simulink model "sparrow_albatros_spec_withgpio_bram"  (R2021a)
settings: Solver=VariableStepDiscrete  StartTime=0.0  StopTime=200000  RelTol=1e-3
undefined symbols (not defined in the file): pfb_coeff_gen_calc
libraries: xbsIndex_r4 x5629, casper_library_misc x33, casper_library_delays x28, xps_library x10, simulink x8, xbsReplacements_r4 x2
(part 5 of 85)

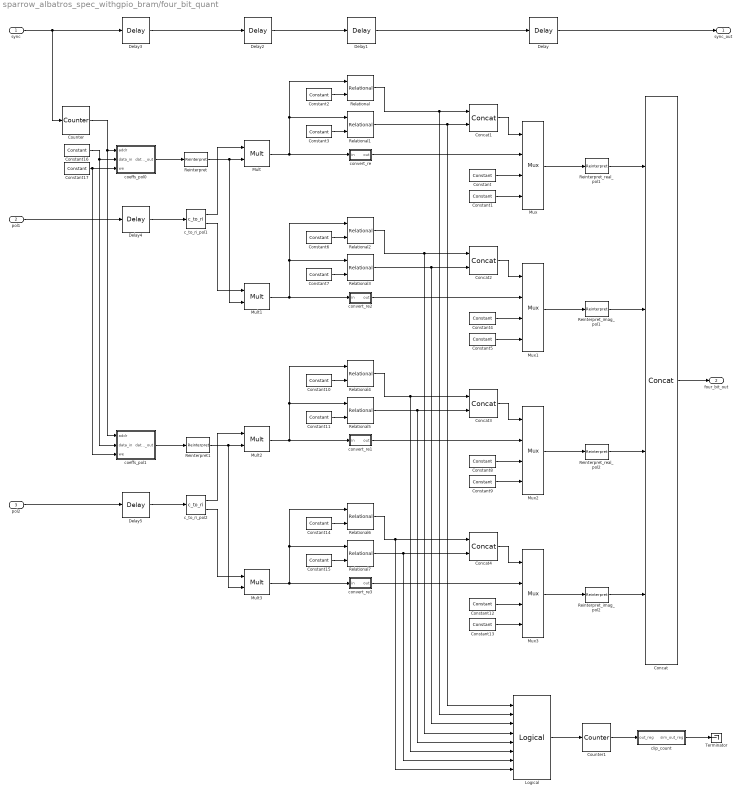
== system sparrow_albatros_spec_withgpio_bram/four_bit_quant ==
  sync : Inport
  pol1 : Inport  Port=2
  pol2 : Inport  Port=3
  Concat : xbsIndex_r4/Concat  num_inputs=4  dbl_ovrd=off  block_type=concat
  Concat{1..4} (4 alike) : xbsIndex_r4/Concat  num_inputs=2  dbl_ovrd=off  block_type=concat
  Constant{,4,8,12} (4 alike) : xbsIndex_r4/Constant  const=7/8  gui_display_data_type=Fixed-point  arith_type=Signed (2's comp)  n_bits=4  bin_pt=3  preci_type=Single  exp_width=8  frac_width=24  explicit_period=on  period=1  equ=P=C  opselect=C  inp2=PCIN>>17  opr=+  inp1=P  carry=CIN  dbl_ovrd=off  block_type=constant
  Constant{1,5,9,13} (4 alike) : xbsIndex_r4/Constant  const=-7/8  gui_display_data_type=Fixed-point  arith_type=Signed (2's comp)  n_bits=4  bin_pt=3  preci_type=Single  exp_width=8  frac_width=24  explicit_period=on  period=1  equ=P=C  opselect=C  inp2=PCIN>>17  opr=+  inp1=P  carry=CIN  dbl_ovrd=off  block_type=constant
  Constant{2,6,10,14} (4 alike) : xbsIndex_r4/Constant  const=-7/8  gui_display_data_type=Fixed-point  arith_type=Signed (2's comp)  n_bits=18  bin_pt=17  preci_type=Single  exp_width=8  frac_width=24  explicit_period=on  period=1  equ=P=C  opselect=C  inp2=PCIN>>17  opr=+  inp1=P  carry=CIN  dbl_ovrd=off  block_type=constant
  Constant{3,7,11,15} (4 alike) : xbsIndex_r4/Constant  const=7/8  gui_display_data_type=Fixed-point  arith_type=Signed (2's comp)  n_bits=18  bin_pt=17  preci_type=Single  exp_width=8  frac_width=24  explicit_period=on  period=1  equ=P=C  opselect=C  inp2=PCIN>>17  opr=+  inp1=P  carry=CIN  dbl_ovrd=off  block_type=constant
  Constant16 : xbsIndex_r4/Constant  const=0  gui_display_data_type=Fixed-point  arith_type=Signed (2's comp)  n_bits=32  bin_pt=0  preci_type=Single  exp_width=8  frac_width=24  explicit_period=on  period=1  equ=P=C  opselect=C  inp2=PCIN>>17  opr=+  inp1=P  carry=CIN  dbl_ovrd=off  block_type=constant
  Constant17 : xbsIndex_r4/Constant  const=0  gui_display_data_type=Boolean  arith_type=Boolean  n_bits=16  bin_pt=14  preci_type=Single  exp_width=8  frac_width=24  explicit_period=on  period=1  equ=P=C  opselect=C  inp2=PCIN>>17  opr=+  inp1=P  carry=CIN  dbl_ovrd=off  block_type=constant
  Counter : xbsIndex_r4/Counter  cnt_type=Free Running  cnt_to=50  operation=Up  start_count=0  cnt_by_val=1  arith_type=Unsigned  n_bits=11  bin_pt=0  load_pin=off  rst=on  en=off  explicit_period=on  period=1  use_behavioral_HDL=off  implementation=Fabric  dbl_ovrd=off  block_type=counter
  Counter1 : xbsIndex_r4/Counter  cnt_type=Free Running  cnt_to=Inf  operation=Up  start_count=0  cnt_by_val=1  arith_type=Unsigned  n_bits=32  bin_pt=0  load_pin=off  rst=off  en=on  explicit_period=on  period=1  use_behavioral_HDL=off  implementation=Fabric  dbl_ovrd=off  block_type=counter
  Delay{,3..5} (4 alike) : xbsIndex_r4/Delay  rst=off  infoeditControl=Selection of Reset will increase slice count due to use of real FFs and instead of SRLs  en=off  latency=1  reg_retiming=off  dbl_ovrd=off  block_type=delay
  Delay1 : xbsIndex_r4/Delay  rst=off  infoeditControl=Selection of Reset will increase slice count due to use of real FFs and instead of SRLs  en=off  latency=2  reg_retiming=off  dbl_ovrd=off  block_type=delay
  Delay2 : xbsIndex_r4/Delay  rst=off  infoeditControl=Selection of Reset will increase slice count due to use of real FFs and instead of SRLs  en=off  latency=3  reg_retiming=off  dbl_ovrd=off  block_type=delay
  Logical : xbsIndex_r4/Logical  logical_function=OR  inputs=8  en=off  latency=1  precision=Full  arith_type=Unsigned  n_bits=16  bin_pt=0  align_bp=on  dbl_ovrd=off  block_type=logical
  Mult{,1..3} (4 alike) : xbsIndex_r4/Mult  precision=Full  arith_type="Signed  (2's comp)"  n_bits=16  bin_pt=14  quantization=Truncate  overflow=Wrap  en=off  latency=3  use_behavioral_HDL=off  opt=Speed  use_embedded=on  optimum_pipeline=off  pipeline=on  dbl_ovrd=off  use_rpm=on  placement_style=Triangular  block_type=mult
  Mux{,1..3} (4 alike) : xbsIndex_r4/Mux  inputs=3  en=off  latency=1  precision=Full  arith_type=Unsigned  n_bits=16  bin_pt=14  quantization=Truncate  overflow=Wrap  dbl_ovrd=off  block_type=mux
  Reinterpret : xbsIndex_r4/Reinterpret  force_arith_type=on  arith_type="Signed  (2's comp)"  force_bin_pt=on  bin_pt=15  block_type=reinterpret
  Reinterpret1 : xbsIndex_r4/Reinterpret  force_arith_type=on  arith_type="Signed  (2's comp)"  force_bin_pt=on  bin_pt=15  block_type=reinterpret
  Reinterpret_imag_pol1 : xbsIndex_r4/Reinterpret  force_arith_type=on  arith_type=Unsigned  force_bin_pt=on  bin_pt=0  block_type=reinterpret
  Reinterpret_imag_pol2 : xbsIndex_r4/Reinterpret  force_arith_type=on  arith_type=Unsigned  force_bin_pt=on  bin_pt=0  block_type=reinterpret
  Reinterpret_real_pol1 : xbsIndex_r4/Reinterpret  force_arith_type=on  arith_type=Unsigned  force_bin_pt=on  bin_pt=0  block_type=reinterpret
  Reinterpret_real_pol2 : xbsIndex_r4/Reinterpret  force_arith_type=on  arith_type=Unsigned  force_bin_pt=on  bin_pt=0  block_type=reinterpret
  Relational{,2,4,6} (4 alike) : xbsIndex_r4/Relational  mode=a<b  op_type=Bool  en=off  latency=2  dbl_ovrd=off  block_type=relational
  Relational{1,3,5,7} (4 alike) : xbsIndex_r4/Relational  mode=a>b  op_type=Bool  en=off  latency=2  dbl_ovrd=off  block_type=relational
  Terminator : Terminator
  c_to_ri_pol1 : casper_library_misc/c_to_ri  n_bits=24  bin_pt=23
      settings: AttributesFormatString=24_23 r/i  SourceProductName=CASPER DSP Blockset
  c_to_ri_pol2 : casper_library_misc/c_to_ri  n_bits=24  bin_pt=23
      settings: AttributesFormatString=24_23 r/i  SourceProductName=CASPER DSP Blockset
  clip_count : Subsystem  Tag=xps:sw_reg  AncestorBlock=xps_library/Memory/software_register  mask(swreg){io_dir=To Processor, io_delay=0, init_val=0, sample_period=1, names=reg, bitwidths=32, bin_pts=0, arith_types=0, sim_port=on, show_format=on}
      mask prompts: io_dir "I/O direction"; io_delay "I/O delay"; init_val "Initial Value"; sample_period "Sample period"; names "Bitfield names [msb...lsb]"; bitwidths "Bitfield widths"; bin_pts "Bitfield binary pts"; arith_types "Bitfield types, ufix=0, fix=1, bool=2"; sim_port "Provide sim input/output?"; show_format "Print format string?"
      mask help: A 32-bit software-accessible register. Can be divided into bitfields of varying widths and types using the fields in the block mask.
      mask init:
      | swreg_init(gcb)
      settings: AttributesFormatString=1output:uf32.0 = 32 bits
      mask TypeOptions io_dir: To Processor | From Processor
      mask Callback io_dir:
      | mask_enables = get_param(gcb, 'MaskEnables');
      | mask_names = get_param(gcb, 'MaskNames');
      | if strcmp(get_param(gcb, 'io_dir'), 'To Processor'),
      |     mask_enables{ismember(mask_names, 'sample_period')} = 'off';
      | else
      |     mask_enables{ismember(mask_names, 'sample_period')} = 'on';
      | end
      | set_param(gcb, 'MaskEnables', mask_enables);
      mask DialogControl ParameterTabVar0 Prompt: Setup
  coeffs_pol0 : Subsystem  Tag=xps:bram  AncestorBlock=xps_library/Memory/shared_bram  mask{arith_type=Unsigned, addr_width=11, data_width=32, reg_prim_output=off, reg_core_output=off, optimization=Minimum_Area, data_bin_pt=0, init_vals=ones(1,2048)*(2^31), sample_rate=1}
      mask prompts: arith_type "Output Data Type"; addr_width "Address width"; data_width "Data Width"; reg_prim_output "Register Primitive Output"; reg_core_output "Register Core Output"; data_bin_pt "Data Binary Point"; init_vals "Initial values (simulation only)"; sample_rate "Sample rate"
      mask init:
      | shared_bram_mask;
      mask TypeOptions arith_type: Unsigned | Signed  (2's comp)
      mask TypeOptions data_width: 8 | 16 | 32 | 64 | 128
      mask TypeOptions optimization: Minimum_Area | Low_Power
  coeffs_pol1 : Subsystem  Tag=xps:bram  AncestorBlock=xps_library/Memory/shared_bram  mask{arith_type=Unsigned, addr_width=11, data_width=32, reg_prim_output=off, reg_core_output=off, optimization=Minimum_Area, data_bin_pt=0, init_vals=ones(1,2048)*(2^31), sample_rate=1}
      mask prompts: arith_type "Output Data Type"; addr_width "Address width"; data_width "Data Width"; reg_prim_output "Register Primitive Output"; reg_core_output "Register Core Output"; data_bin_pt "Data Binary Point"; init_vals "Initial values (simulation only)"; sample_rate "Sample rate"
      mask init:
      | shared_bram_mask;
      mask TypeOptions arith_type: Unsigned | Signed  (2's comp)
      mask TypeOptions data_width: 8 | 16 | 32 | 64 | 128
      mask TypeOptions optimization: Minimum_Area | Low_Power
  convert_re : Subsystem  AncestorBlock=casper_library_misc/convert  mask(convert){bin_pt_in=38, n_bits_out=4, bin_pt_out=3, quantization=Round  (unbiased: Even Values), overflow=Wrap, csp_latency=2}
      mask prompts: bin_pt_in "Binary Point In"; n_bits_out "Bit Width Out"; bin_pt_out "Binary Point Out"; csp_latency "Latency"
      mask help:
      | Convert input value to the specified bit width and precision.
      |
      | Does not support upscaling number of fractional bits (eg 8_5 to 8_4 is ok, but not 8_4 to 8_5).
      mask init:
      | convert_init(gcb, ...
      |     'bin_pt_in',bin_pt_in, ...
      |     'n_bits_out',n_bits_out,...
      |     'bin_pt_out',bin_pt_out, ...
      |     'quantization',quantization,...
      |     'overflow',overflow,...
      |     'csp_latency',csp_latency);
      settings: AttributesFormatString=|
      | N_38 ==> 4_3
      | round even, wrap
      | latency = 2
      mask Help:
      | <pre>
      | Description::
      | 
      | Outputs converted version of the input.
      | 
      | Mask Parameters::
      | 
      | Binary Point In (bin_pt_in): Specifies the binary point location in the input.
      | 
      | Bit Width Out (n_bits_out): Specifies the width of the output.
      | 
      | Binary Point Out (bin_pt_out): Specifies the binary point location in the output.
      | 
      | Quantization (quantization): Specifies quantization handling.
      | 
      | Overflow (overflow): Specifies overflow handling.
      | 
      | Latency (latency): Specifies the latency of the underlying adder block, which is the overall
      | latency of this block as well.
      | </pre>
      mask TypeOptions quantization: Truncate | Round  (unbiased: +/- Inf) | Round  (unbiased: Even Values) | Round  (unbiased: Zero) | Round  (unbiased: Odd Values) | Round  (biased: Up) | Round  (biased: Down)
      mask TypeOptions overflow: Wrap | Saturate | Error
  convert_re1 : Subsystem  AncestorBlock=casper_library_misc/convert  mask(convert){bin_pt_in=38, n_bits_out=4, bin_pt_out=3, quantization=Round  (unbiased: Even Values), overflow=Wrap, csp_latency=2}
      mask prompts: bin_pt_in "Binary Point In"; n_bits_out "Bit Width Out"; bin_pt_out "Binary Point Out"; csp_latency "Latency"
      mask help:
      | Convert input value to the specified bit width and precision.
      |
      | Does not support upscaling number of fractional bits (eg 8_5 to 8_4 is ok, but not 8_4 to 8_5).
      mask init: same as sparrow_albatros_spec_withgpio_bram/four_bit_quant/convert_re
      settings: AttributesFormatString=|
      | N_38 ==> 4_3
      | round even, wrap
      | latency = 2
      mask Help:
      | <pre>
      | Description::
      | 
      | Outputs converted version of the input.
      | 
      | Mask Parameters::
      | 
      | Binary Point In (bin_pt_in): Specifies the binary point location in the input.
      | 
      | Bit Width Out (n_bits_out): Specifies the width of the output.
      | 
      | Binary Point Out (bin_pt_out): Specifies the binary point location in the output.
      | 
      | Quantization (quantization): Specifies quantization handling.
      | 
      | Overflow (overflow): Specifies overflow handling.
      | 
      | Latency (latency): Specifies the latency of the underlying adder block, which is the overall
      | latency of this block as well.
      | </pre>
      mask TypeOptions quantization: Truncate | Round  (unbiased: +/- Inf) | Round  (unbiased: Even Values) | Round  (unbiased: Zero) | Round  (unbiased: Odd Values) | Round  (biased: Up) | Round  (biased: Down)
      mask TypeOptions overflow: Wrap | Saturate | Error
  convert_re2 : Subsystem  AncestorBlock=casper_library_misc/convert  mask(convert){bin_pt_in=38, n_bits_out=4, bin_pt_out=3, quantization=Round  (unbiased: Even Values), overflow=Wrap, csp_latency=2}
      mask prompts: bin_pt_in "Binary Point In"; n_bits_out "Bit Width Out"; bin_pt_out "Binary Point Out"; csp_latency "Latency"
      mask help:
      | Convert input value to the specified bit width and precision.
      |
      | Does not support upscaling number of fractional bits (eg 8_5 to 8_4 is ok, but not 8_4 to 8_5).
      mask init: same as sparrow_albatros_spec_withgpio_bram/four_bit_quant/convert_re
      settings: AttributesFormatString=|
      | N_38 ==> 4_3
      | round even, wrap
      | latency = 2
      mask Help:
      | <pre>
      | Description::
      | 
      | Outputs converted version of the input.
      | 
      | Mask Parameters::
      | 
      | Binary Point In (bin_pt_in): Specifies the binary point location in the input.
      | 
      | Bit Width Out (n_bits_out): Specifies the width of the output.
      | 
      | Binary Point Out (bin_pt_out): Specifies the binary point location in the output.
      | 
      | Quantization (quantization): Specifies quantization handling.
      | 
      | Overflow (overflow): Specifies overflow handling.
      | 
      | Latency (latency): Specifies the latency of the underlying adder block, which is the overall
      | latency of this block as well.
      | </pre>
      mask TypeOptions quantization: Truncate | Round  (unbiased: +/- Inf) | Round  (unbiased: Even Values) | Round  (unbiased: Zero) | Round  (unbiased: Odd Values) | Round  (biased: Up) | Round  (biased: Down)
      mask TypeOptions overflow: Wrap | Saturate | Error
  convert_re3 : Subsystem  AncestorBlock=casper_library_misc/convert  mask(convert){bin_pt_in=38, n_bits_out=4, bin_pt_out=3, quantization=Round  (unbiased: Even Values), overflow=Wrap, csp_latency=2}
      mask prompts: bin_pt_in "Binary Point In"; n_bits_out "Bit Width Out"; bin_pt_out "Binary Point Out"; csp_latency "Latency"
      mask help:
      | Convert input value to the specified bit width and precision.
      |
      | Does not support upscaling number of fractional bits (eg 8_5 to 8_4 is ok, but not 8_4 to 8_5).
      mask init: same as sparrow_albatros_spec_withgpio_bram/four_bit_quant/convert_re
      settings: AttributesFormatString=|
      | N_38 ==> 4_3
      | round even, wrap
      | latency = 2
      mask Help:
      | <pre>
      | Description::
      | 
      | Outputs converted version of the input.
      | 
      | Mask Parameters::
      | 
      | Binary Point In (bin_pt_in): Specifies the binary point location in the input.
      | 
      | Bit Width Out (n_bits_out): Specifies the width of the output.
      | 
      | Binary Point Out (bin_pt_out): Specifies the binary point location in the output.
      | 
      | Quantization (quantization): Specifies quantization handling.
      | 
      | Overflow (overflow): Specifies overflow handling.
      | 
      | Latency (latency): Specifies the latency of the underlying adder block, which is the overall
      | latency of this block as well.
      | </pre>
      mask TypeOptions quantization: Truncate | Round  (unbiased: +/- Inf) | Round  (unbiased: Even Values) | Round  (unbiased: Zero) | Round  (unbiased: Odd Values) | Round  (biased: Up) | Round  (biased: Down)
      mask TypeOptions overflow: Wrap | Saturate | Error
  sync_out : Outport  VectorParamsAs1DForOutWhenUnconnected=off
  four_bit_out : Outport  Port=2  VectorParamsAs1DForOutWhenUnconnected=off
  wires:
  Delay5/1 -> c_to_ri_pol2/1
  Delay4/1 -> c_to_ri_pol1/1
  Delay3/1 -> Delay2/1
  coeffs_pol0/1(data_out) -> Reinterpret/1
  Delay2/1 -> Delay1/1
  Delay1/1 -> Delay/1
  Delay/1 -> sync_out/1
  Mux3/1 -> Reinterpret_imag_pol2/1
  Mux2/1 -> Reinterpret_real_pol2/1
  c_to_ri_pol2/2 -> Mult3/1
  c_to_ri_pol2/1 -> Mult2/1
  Mult3/1 -> convert_re3/1(in), Relational7/1, Relational6/1
  Constant14/1 -> Relational6/2
  Constant15/1 -> Relational7/2
  Relational7/1 -> Concat4/2, Logical/7
  Relational6/1 -> Logical/8, Concat4/1
  Concat4/1 -> Mux3/1
  convert_re3/1(out) -> Mux3/2
  Constant13/1 -> Mux3/4
  Constant12/1 -> Mux3/3
  Mult2/1 -> convert_re1/1(in), Relational5/1, Relational4/1
  Constant10/1 -> Relational4/2
  Constant11/1 -> Relational5/2
  Relational5/1 -> Concat3/2, Logical/5
  Relational4/1 -> Concat3/1, Logical/6
  Concat3/1 -> Mux2/1
  convert_re1/1(out) -> Mux2/2
  Constant9/1 -> Mux2/4
  Constant8/1 -> Mux2/3
  pol2/1 -> Delay5/1
  c_to_ri_pol1/2 -> Mult1/1
  c_to_ri_pol1/1 -> Mult/1
  Mux1/1 -> Reinterpret_imag_pol1/1
  Mult1/1 -> convert_re2/1(in), Relational3/1, Relational2/1
  Constant6/1 -> Relational2/2
  Constant7/1 -> Relational3/2
  Relational3/1 -> Concat2/2, Logical/3
  Relational2/1 -> Concat2/1, Logical/4
  Concat2/1 -> Mux1/1
  convert_re2/1(out) -> Mux1/2
  Constant5/1 -> Mux1/4
  Constant4/1 -> Mux1/3
  Mult/1 -> convert_re/1(in), Relational1/1, Relational/1
  Constant2/1 -> Relational/2
  Constant3/1 -> Relational1/2
  Relational1/1 -> Concat1/2, Logical/1
  Relational/1 -> Concat1/1, Logical/2
  Concat1/1 -> Mux/1
  convert_re/1(out) -> Mux/2
  Constant1/1 -> Mux/4
  Constant/1 -> Mux/3
  Mux/1 -> Reinterpret_real_pol1/1
  Reinterpret_real_pol2/1 -> Concat/3
  pol1/1 -> Delay4/1
  Reinterpret_imag_pol1/1 -> Concat/2
  Reinterpret_imag_pol2/1 -> Concat/4
  Concat/1 -> four_bit_out/1
  Reinterpret_real_pol1/1 -> Concat/1
  Constant17/1 -> coeffs_pol1/3(we), coeffs_pol0/3(we)
  Constant16/1 -> coeffs_pol1/2(data_in), coeffs_pol0/2(data_in)
  Counter/1 -> coeffs_pol1/1(addr), coeffs_pol0/1(addr)
  sync/1 -> Counter/1, Delay3/1
  clip_count/1(sim_out_reg) -> Terminator/1
  Logical/1 -> Counter1/1
  Counter1/1 -> clip_count/1(out_reg)
  Reinterpret/1 -> Mult1/2, Mult/2
  coeffs_pol1/1(data_out) -> Reinterpret1/1
  Reinterpret1/1 -> Mult3/2, Mult2/2

== system sparrow_albatros_spec_withgpio_bram/four_bit_reorder ==
  note: always high
  note: delay over this block is truly 2048, ignore the z-1 or block doesn't change logic, is high
  note: a delay to account for the counter starting
  note: starts counting on clk#1
      | i.e. counter at 1 on clk#2
  sync_in : Inport
  d_in : Inport  Port=2
  Constant2 : xbsIndex_r4/Constant  const=1  gui_display_data_type=Boolean  arith_type=Boolean  n_bits=8  bin_pt=0  preci_type=Single  exp_width=8  frac_width=24  explicit_period=on  period=1  equ=P=C  opselect=C  inp2=PCIN>>17  opr=+  inp1=P  carry=CIN  dbl_ovrd=off  block_type=constant
  Counter1 : xbsIndex_r4/Counter  cnt_type=Free Running  cnt_to=Inf  operation=Up  start_count=0  cnt_by_val=1  arith_type=Unsigned  n_bits=12  bin_pt=0  load_pin=off  rst=on  en=off  explicit_period=on  period=1  use_behavioral_HDL=on  implementation=Fabric  dbl_ovrd=off  block_type=counter
  Scope1 : Scope  NumInputPorts=4
  Slice1 : xbsIndex_r4/Slice  nbits=1  boolean_output=off  mode=Upper Bit Location + Width  bit1=0  base1=MSB of Input  bit0=0  base0=LSB of Input  dbl_ovrd=off  block_type=slice
  Slice2 : xbsIndex_r4/Slice  nbits=11  boolean_output=off  mode=Lower Bit Location + Width  bit1=0  base1=MSB of Input  bit0=0  base0=LSB of Input  dbl_ovrd=off  block_type=slice
  data_out : xbsIndex_r4/Gateway Out  inherit_from_input=off  hdl_port=on  rows=1  columns=1  UseAsDAC=off  DACChannel='1'  interface=None  automatic_assignment=on  address_offset=hex2dec('00')  intf_name=''  intf_description=''  timing_constraint=None  locs_specified=off  LOCs={}  io_standard={}  block_type=gatewayout
  dbl_buffer0 : Subsystem  AncestorBlock=casper_library_reorder/dbl_buffer  mask(dbl_buffer){depth=2048, csp_latency=2}
      mask prompts: csp_latency "Latency"
  delay_d0 : xbsIndex_r4/Delay  rst=off  infoeditControl=Selection of Reset will increase slice count due to use of real FFs and instead of SRLs  en=off  latency=3  reg_retiming=on  dbl_ovrd=off  block_type=delay
  delay_din0 : xbsIndex_r4/Delay  rst=off  infoeditControl=Selection of Reset will increase slice count due to use of real FFs and instead of SRLs  en=off  latency=3  reg_retiming=on  dbl_ovrd=off  block_type=delay
  delay_sel : xbsIndex_r4/Delay  rst=off  infoeditControl=Selection of Reset will increase slice count due to use of real FFs and instead of SRLs  en=off  latency=3  reg_retiming=on  dbl_ovrd=off  block_type=delay
  din : xbsIndex_r4/Gateway Out  inherit_from_input=off  hdl_port=on  rows=1  columns=1  UseAsDAC=off  DACChannel='1'  interface=None  automatic_assignment=on  address_offset=hex2dec('00')  intf_name=''  intf_description=''  timing_constraint=None  locs_specified=off  LOCs={}  io_standard={}  block_type=gatewayout
  map : xbsIndex_r4/Gateway Out  inherit_from_input=off  hdl_port=on  rows=1  columns=1  UseAsDAC=off  DACChannel='1'  interface=None  automatic_assignment=on  address_offset=hex2dec('00')  intf_name=''  intf_description=''  timing_constraint=None  locs_specified=off  LOCs={}  io_standard={}  block_type=gatewayout
  map1 : Subsystem  Tag=xps:bram  AncestorBlock=xps_library/Memory/shared_bram  mask{arith_type=Unsigned, addr_width=11, data_width=16, reg_prim_output=on, reg_core_output=on, optimization=Minimum_Area, data_bin_pt=0, init_vals=[40, 0, 41, 0, 42, 0, 43, 0, 44, 0, 45, 0, 46, 0, 47, 0, zeros(1,2048-16)], sample_rate=1}
      mask prompts: arith_type "Output Data Type"; addr_width "Address width"; data_width "Data Width"; reg_prim_output "Register Primitive Output"; reg_core_output "Register Core Output"; data_bin_pt "Data Binary Point"; init_vals "Initial values (simulation only)"; sample_rate "Sample rate"
      mask init:
      | shared_bram_mask;
      mask TypeOptions arith_type: Unsigned | Signed  (2's comp)
      mask TypeOptions data_width: 8 | 16 | 32 | 64 | 128
      mask TypeOptions optimization: Minimum_Area | Low_Power
  never : xbsIndex_r4/Constant  const=0  gui_display_data_type=Fixed-point  arith_type=Boolean  n_bits=16  bin_pt=14  preci_type=Single  exp_width=8  frac_width=24  explicit_period=on  period=1  equ=P=C  opselect=C  inp2=PCIN>>17  opr=+  inp1=P  carry=CIN  dbl_ovrd=off  block_type=constant
  post_sync_delay : xbsIndex_r4/Delay  rst=off  infoeditControl=Selection of Reset will increase slice count due to use of real FFs and instead of SRLs  en=off  latency=4  reg_retiming=on  dbl_ovrd=off  block_type=delay
  post_sync_delay1 : xbsIndex_r4/Delay  rst=off  infoeditControl=Selection of Reset will increase slice count due to use of real FFs and instead of SRLs  en=off  latency=2048  reg_retiming=on  dbl_ovrd=off  block_type=delay
  pre_sync_delay : xbsIndex_r4/Delay  rst=off  infoeditControl=Selection of Reset will increase slice count due to use of real FFs and instead of SRLs  en=off  latency=3  reg_retiming=on  dbl_ovrd=off  block_type=delay
  sw_bram_slice : xbsIndex_r4/Slice  nbits=11  boolean_output=off  mode=Lower Bit Location + Width  bit1=0  base1=MSB of Input  bit0=0  base0=LSB of Input  dbl_ovrd=off  block_type=slice
  syncout1 : xbsIndex_r4/Gateway Out  inherit_from_input=off  hdl_port=on  rows=1  columns=1  UseAsDAC=off  DACChannel='1'  interface=None  automatic_assignment=on  address_offset=hex2dec('00')  intf_name=''  intf_description=''  timing_constraint=None  locs_specified=off  LOCs={}  io_standard={}  block_type=gatewayout
  zero : xbsIndex_r4/Constant  const=0  gui_display_data_type=Fixed-point  arith_type=Unsigned  n_bits=16  bin_pt=0  preci_type=Single  exp_width=8  frac_width=24  explicit_period=on  period=1  equ=P=C  opselect=C  inp2=PCIN>>17  opr=+  inp1=P  carry=CIN  dbl_ovrd=off  block_type=constant
  sync_out : Outport
  dout : Outport  Port=2
  wires:
  zero/1 -> map1/2(data_in)
  syncout1/1 -> Scope1/1
  sync_in/1 -> pre_sync_delay/1, Counter1/1
  sw_bram_slice/1 -> map/1, dbl_buffer0/3(rd_addr)
  map1/1(data_out) -> sw_bram_slice/1
  delay_sel/1 -> dbl_buffer0/1(rw_mode)
  Constant2/1 -> dbl_buffer0/5(we)
  din/1 -> Scope1/2
  Counter1/1 -> Slice2/1, Slice1/1
  post_sync_delay1/1 -> post_sync_delay/1
  data_out/1 -> Scope1/4
  delay_d0/1 -> dbl_buffer0/2(wr_addr)
  delay_din0/1 -> din/1, dbl_buffer0/4(din1)
  pre_sync_delay/1 -> post_sync_delay1/1
  Slice1/1 -> delay_sel/1
  map/1 -> Scope1/3
  post_sync_delay/1 -> sync_out/1, syncout1/1
  never/1 -> map1/3(we)
  d_in/1 -> delay_din0/1
  Slice2/1 -> delay_d0/1, map1/1(addr)
  dbl_buffer0/1(dout) -> dout/1, data_out/1

== system sparrow_albatros_spec_withgpio_bram/gbe_en ==
  sim_1 : Inport
  convert1_1 : DataTypeConversion  OutDataTypeStr=fixdt('ufix1_En0')  LockScale=on
  convert2_1 : DataTypeConversion  OutDataTypeStr=fixdt('ufix1_En0')  ConvertRealWorld=Stored Integer (SI)  LockScale=on
  gain_1 : Gain  OutDataTypeStr=fixdt('ufix32_En0')
  io_delay : xbsIndex_r4/Delay  rst=off  infoeditControl=Selection of Reset will increase slice count due to use of real FFs and instead of SRLs  en=off  latency=0  reg_retiming=on  dbl_ovrd=off  block_type=delay
  slice_reg : xbsIndex_r4/Slice  nbits=1  boolean_output=on  mode=Lower Bit Location + Width  bit1=0  base1=MSB of Input  bit0=0  base0=LSB of Input  dbl_ovrd=off  block_type=slice
  sparrow_albatros_spec_withgpio_bram_gbe_en_user_data_out : xbsIndex_r4/Gateway In  gui_display_data_type=Fixed-point  arith_type=Unsigned  n_bits=32  bin_pt=0  preci_type=Single  exp_width=8  frac_width=24  rows=1  columns=1  quantization="Round  (unbiased: +/- Inf)"  overflow=Saturate  period=1  UseAsADC=off  ADCChannel='1'  interface=None  automatic_assignment=on  address_offset=hex2dec('00')  intf_name=''  intf_description=''  default_value=0  timing_constraint=None  locs_specified=off  LOCs={}  io_standard={}  inherit_from_input=off  hdl_port=on  dbl_ovrd=off  block_type=gatewayin
  in_reg : Outport
  wires:
  sparrow_albatros_spec_withgpio_bram_gbe_en_user_data_out/1 -> io_delay/1
  sim_1/1 -> convert1_1/1
  convert1_1/1 -> convert2_1/1
  convert2_1/1 -> gain_1/1
  gain_1/1 -> sparrow_albatros_spec_withgpio_bram_gbe_en_user_data_out/1
  io_delay/1 -> slice_reg/1
  slice_reg/1 -> in_reg/1

== system sparrow_albatros_spec_withgpio_bram/gbe_rst ==
  sim_1 : Inport
  convert1_1 : DataTypeConversion  OutDataTypeStr=fixdt('ufix1_En0')  LockScale=on
  convert2_1 : DataTypeConversion  OutDataTypeStr=fixdt('ufix1_En0')  ConvertRealWorld=Stored Integer (SI)  LockScale=on
  gain_1 : Gain  OutDataTypeStr=fixdt('ufix32_En0')
  io_delay : xbsIndex_r4/Delay  rst=off  infoeditControl=Selection of Reset will increase slice count due to use of real FFs and instead of SRLs  en=off  latency=0  reg_retiming=on  dbl_ovrd=off  block_type=delay
  reint1 : xbsIndex_r4/Reinterpret  force_arith_type=on  arith_type=Unsigned  force_bin_pt=on  bin_pt=0  block_type=reinterpret
  slice_reg : xbsIndex_r4/Slice  nbits=1  boolean_output=off  mode=Lower Bit Location + Width  bit1=0  base1=MSB of Input  bit0=0  base0=LSB of Input  dbl_ovrd=off  block_type=slice
  sparrow_albatros_spec_withgpio_bram_gbe_rst_user_data_out : xbsIndex_r4/Gateway In  gui_display_data_type=Fixed-point  arith_type=Unsigned  n_bits=32  bin_pt=0  preci_type=Single  exp_width=8  frac_width=24  rows=1  columns=1  quantization="Round  (unbiased: +/- Inf)"  overflow=Saturate  period=1  UseAsADC=off  ADCChannel='1'  interface=None  automatic_assignment=on  address_offset=hex2dec('00')  intf_name=''  intf_description=''  default_value=0  timing_constraint=None  locs_specified=off  LOCs={}  io_standard={}  inherit_from_input=off  hdl_port=on  dbl_ovrd=off  block_type=gatewayin
  in_reg : Outport
  wires:
  sparrow_albatros_spec_withgpio_bram_gbe_rst_user_data_out/1 -> io_delay/1
  sim_1/1 -> convert1_1/1
  convert1_1/1 -> convert2_1/1
  convert2_1/1 -> gain_1/1
  gain_1/1 -> sparrow_albatros_spec_withgpio_bram_gbe_rst_user_data_out/1
  io_delay/1 -> slice_reg/1
  slice_reg/1 -> reint1/1
  reint1/1 -> in_reg/1

== system sparrow_albatros_spec_withgpio_bram/gpio_dsub ==
  sim_1 : Inport
  convert1_1 : DataTypeConversion  OutDataTypeStr=fixdt('ufix32_En0')  LockScale=on
  convert2_1 : DataTypeConversion  OutDataTypeStr=fixdt('ufix32_En0')  ConvertRealWorld=Stored Integer (SI)  LockScale=on
  gain_1 : Gain  OutDataTypeStr=fixdt('ufix32_En0')
  io_delay : xbsIndex_r4/Delay  rst=off  infoeditControl=Selection of Reset will increase slice count due to use of real FFs and instead of SRLs  en=off  latency=0  reg_retiming=on  dbl_ovrd=off  block_type=delay
  reint1 : xbsIndex_r4/Reinterpret  force_arith_type=on  arith_type=Unsigned  force_bin_pt=on  bin_pt=0  block_type=reinterpret
  slice_reg : xbsIndex_r4/Slice  nbits=32  boolean_output=off  mode=Lower Bit Location + Width  bit1=0  base1=MSB of Input  bit0=0  base0=LSB of Input  dbl_ovrd=off  block_type=slice
  sparrow_albatros_spec_withgpio_bram_gpio_dsub_user_data_out : xbsIndex_r4/Gateway In  gui_display_data_type=Fixed-point  arith_type=Unsigned  n_bits=32  bin_pt=0  preci_type=Single  exp_width=8  frac_width=24  rows=1  columns=1  quantization="Round  (unbiased: +/- Inf)"  overflow=Saturate  period=1  UseAsADC=off  ADCChannel='1'  interface=None  automatic_assignment=on  address_offset=hex2dec('00')  intf_name=''  intf_description=''  default_value=0  timing_constraint=None  locs_specified=off  LOCs={}  io_standard={}  inherit_from_input=off  hdl_port=on  dbl_ovrd=off  block_type=gatewayin
  in_reg : Outport
  wires:
  sparrow_albatros_spec_withgpio_bram_gpio_dsub_user_data_out/1 -> io_delay/1
  sim_1/1 -> convert1_1/1
  convert1_1/1 -> convert2_1/1
  convert2_1/1 -> gain_1/1
  gain_1/1 -> sparrow_albatros_spec_withgpio_bram_gpio_dsub_user_data_out/1
  io_delay/1 -> slice_reg/1
  slice_reg/1 -> reint1/1
  reint1/1 -> in_reg/1

== system sparrow_albatros_spec_withgpio_bram/gpio_led_counter ==
  out_reg : Inport
  assert_reg : xbsIndex_r4/Assert  assert_type=on  type_source=Explicitly  gui_display_data_type=Fixed-point  arith_type=Unsigned  n_bits=27  bin_pt=0  preci_type=Single  exp_width=8  frac_width=24  assert_rate=off  rate_source=Explicitly  period=1  output_port=on  block_type=assert
  cast_gw : xbsIndex_r4/Convert  gui_display_data_type=Fixed-point  arith_type=Unsigned  n_bits=32  bin_pt=0  float_type=Single  exp_bits=8  fraction_bits=24  quantization=Truncate  overflow=Wrap  en=off  latency=1  pipeline=off  dbl_ovrd=off  block_type=convert
  io_delay : xbsIndex_r4/Delay  rst=off  infoeditControl=Selection of Reset will increase slice count due to use of real FFs and instead of SRLs  en=off  latency=0  reg_retiming=on  dbl_ovrd=off  block_type=delay
  reint1 : xbsIndex_r4/Reinterpret  force_arith_type=on  arith_type=Unsigned  force_bin_pt=on  bin_pt=0  block_type=reinterpret
  sim_out : Terminator
  sim_out_reg_gw : xbsIndex_r4/Gateway Out  inherit_from_input=off  hdl_port=off  rows=1  columns=1  UseAsDAC=off  DACChannel='1'  interface=None  automatic_assignment=on  address_offset=hex2dec('00')  intf_name=''  intf_description=''  timing_constraint=None  locs_specified=off  LOCs={}  io_standard={}  block_type=gatewayout
  sim_out_reg_sim_delay : xbsIndex_r4/Delay  rst=off  infoeditControl=Selection of Reset will increase slice count due to use of real FFs and instead of SRLs  en=off  latency=1  reg_retiming=on  dbl_ovrd=off  block_type=delay
  sparrow_albatros_spec_withgpio_bram_gpio_led_counter_user_data_in : xbsIndex_r4/Gateway Out  inherit_from_input=off  hdl_port=on  rows=1  columns=1  UseAsDAC=off  DACChannel='1'  interface=None  automatic_assignment=on  address_offset=hex2dec('00')  intf_name=''  intf_description=''  timing_constraint=None  locs_specified=off  LOCs={}  io_standard={}  block_type=gatewayout
  sim_out_reg : Outport
  wires:
  sim_out_reg_sim_delay/1 -> sim_out_reg_gw/1
  sim_out_reg_gw/1 -> sim_out_reg/1
  io_delay/1 -> cast_gw/1
  cast_gw/1 -> sparrow_albatros_spec_withgpio_bram_gpio_led_counter_user_data_in/1
  sparrow_albatros_spec_withgpio_bram_gpio_led_counter_user_data_in/1 -> sim_out/1
  out_reg/1 -> sim_out_reg_sim_delay/1, assert_reg/1
  assert_reg/1 -> reint1/1
  reint1/1 -> io_delay/1

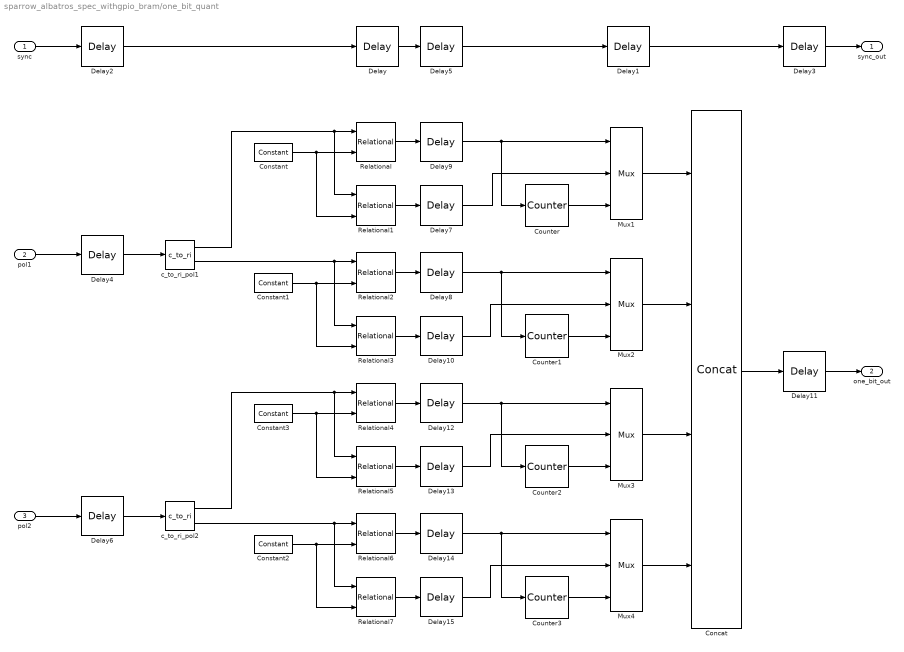
== system sparrow_albatros_spec_withgpio_bram/one_bit_quant ==
  sync : Inport
  pol1 : Inport  Port=2
  pol2 : Inport  Port=3
  Concat : xbsIndex_r4/Concat  num_inputs=4  dbl_ovrd=off  block_type=concat
  Constant{,1..3} (4 alike) : xbsIndex_r4/Constant  const=0  gui_display_data_type=Fixed-point  arith_type=Signed (2's comp)  n_bits=24  bin_pt=23  preci_type=Single  exp_width=8  frac_width=24  explicit_period=on  period=1  equ=P=C  opselect=C  inp2=PCIN>>17  opr=+  inp1=P  carry=CIN  dbl_ovrd=off  block_type=constant
  Counter{,1..3} (4 alike) : xbsIndex_r4/Counter  cnt_type=Free Running  cnt_to=1  operation=Up  start_count=0  cnt_by_val=1  arith_type=Unsigned  n_bits=1  bin_pt=0  load_pin=off  rst=off  en=on  explicit_period=on  period=1  use_behavioral_HDL=off  implementation=Fabric  dbl_ovrd=off  block_type=counter
  Delay{,1..2,4..10,12..15} (14 alike) : xbsIndex_r4/Delay  rst=off  infoeditControl=Selection of Reset will increase slice count due to use of real FFs and instead of SRLs  en=off  latency=2  reg_retiming=off  dbl_ovrd=off  block_type=delay
  Delay11 : xbsIndex_r4/Delay  rst=off  infoeditControl=Selection of Reset will increase slice count due to use of real FFs and instead of SRLs  en=off  latency=1  reg_retiming=off  dbl_ovrd=off  block_type=delay
  Delay3 : xbsIndex_r4/Delay  rst=off  infoeditControl=Selection of Reset will increase slice count due to use of real FFs and instead of SRLs  en=off  latency=1  reg_retiming=off  dbl_ovrd=off  block_type=delay
  Mux{1..4} (4 alike) : xbsIndex_r4/Mux  inputs=2  en=off  latency=2  precision=Full  arith_type=Unsigned  n_bits=16  bin_pt=14  quantization=Truncate  overflow=Wrap  dbl_ovrd=off  block_type=mux
  Relational{,2,4,6} (4 alike) : xbsIndex_r4/Relational  mode=a=b  op_type=Bool  en=off  latency=2  dbl_ovrd=off  block_type=relational
  Relational{1,3,5,7} (4 alike) : xbsIndex_r4/Relational  mode=a>b  op_type=Ufix  en=off  latency=2  dbl_ovrd=off  block_type=relational
  c_to_ri_pol1 : casper_library_misc/c_to_ri  n_bits=24  bin_pt=23
      settings: AttributesFormatString=24_23 r/i  SourceProductName=CASPER DSP Blockset
  c_to_ri_pol2 : casper_library_misc/c_to_ri  n_bits=24  bin_pt=23
      settings: AttributesFormatString=24_23 r/i  SourceProductName=CASPER DSP Blockset
  sync_out : Outport  VectorParamsAs1DForOutWhenUnconnected=off
  one_bit_out : Outport  Port=2  VectorParamsAs1DForOutWhenUnconnected=off
  wires:
  Mux4/1 -> Concat/4
  sync/1 -> Delay2/1
  Mux2/1 -> Concat/2
  Delay/1 -> Delay5/1
  Delay1/1 -> Delay3/1
  c_to_ri_pol1/1 -> Relational1/1, Relational/1
  Mux1/1 -> Concat/1
  Counter/1 -> Mux1/3
  Mux3/1 -> Concat/3
  Constant/1 -> Relational/2, Relational1/2
  c_to_ri_pol1/2 -> Relational2/1, Relational3/1
  Counter1/1 -> Mux2/3
  Constant1/1 -> Relational3/2, Relational2/2
  c_to_ri_pol2/1 -> Relational4/1, Relational5/1
  Counter2/1 -> Mux3/3
  Constant3/1 -> Relational5/2, Relational4/2
  Relational7/1 -> Delay15/1
  c_to_ri_pol2/2 -> Relational7/1, Relational6/1
  Counter3/1 -> Mux4/3
  Constant2/1 -> Relational6/2, Relational7/2
  Delay2/1 -> Delay/1
  pol1/1 -> Delay4/1
  pol2/1 -> Delay6/1
  Relational/1 -> Delay9/1
  Delay5/1 -> Delay1/1
  Relational1/1 -> Delay7/1
  Relational2/1 -> Delay8/1
  Relational3/1 -> Delay10/1
  Relational4/1 -> Delay12/1
  Relational5/1 -> Delay13/1
  Relational6/1 -> Delay14/1
  Delay15/1 -> Mux4/2
  Concat/1 -> Delay11/1
  Delay3/1 -> sync_out/1
  Delay4/1 -> c_to_ri_pol1/1
  Delay6/1 -> c_to_ri_pol2/1
  Delay7/1 -> Mux1/2
  Delay8/1 -> Counter1/1, Mux2/1
  Delay9/1 -> Counter/1, Mux1/1
  Delay10/1 -> Mux2/2
  Delay11/1 -> one_bit_out/1
  Delay12/1 -> Counter2/1, Mux3/1
  Delay13/1 -> Mux3/2
  Delay14/1 -> Counter3/1, Mux4/1

== system sparrow_albatros_spec_withgpio_bram/one_bit_reorder ==
  note: msb 1 bit
  note: lsb 11 bits
  note: super simple, read and write select, explains sync_delay by 2048
  note: 12 bit counter
      | unsigned
  note: delay 3
  sync : Inport
  din0 : Inport  Port=2
  Constant2 : xbsIndex_r4/Constant  const=1  gui_display_data_type=Boolean  arith_type=Boolean  n_bits=8  bin_pt=0  preci_type=Single  exp_width=8  frac_width=24  explicit_period=on  period=1  equ=P=C  opselect=C  inp2=PCIN>>17  opr=+  inp1=P  carry=CIN  dbl_ovrd=off  block_type=constant
  Counter1 : xbsIndex_r4/Counter  cnt_type=Free Running  cnt_to=Inf  operation=Up  start_count=0  cnt_by_val=1  arith_type=Unsigned  n_bits=12  bin_pt=0  load_pin=off  rst=on  en=off  explicit_period=on  period=1  use_behavioral_HDL=on  implementation=Fabric  dbl_ovrd=off  block_type=counter
  Slice1 : xbsIndex_r4/Slice  nbits=1  boolean_output=off  mode=Upper Bit Location + Width  bit1=0  base1=MSB of Input  bit0=0  base0=LSB of Input  dbl_ovrd=off  block_type=slice
  Slice2 : xbsIndex_r4/Slice  nbits=11  boolean_output=off  mode=Lower Bit Location + Width  bit1=0  base1=MSB of Input  bit0=0  base0=LSB of Input  dbl_ovrd=off  block_type=slice
  dbl_buffer0 : Subsystem  AncestorBlock=casper_library_reorder/dbl_buffer  mask(dbl_buffer){depth=2048, csp_latency=2}
      mask prompts: csp_latency "Latency"
  delay_d0 : xbsIndex_r4/Delay  rst=off  infoeditControl=Selection of Reset will increase slice count due to use of real FFs and instead of SRLs  en=off  latency=3  reg_retiming=on  dbl_ovrd=off  block_type=delay
  delay_din0 : xbsIndex_r4/Delay  rst=off  infoeditControl=Selection of Reset will increase slice count due to use of real FFs and instead of SRLs  en=off  latency=3  reg_retiming=on  dbl_ovrd=off  block_type=delay
  delay_sel : xbsIndex_r4/Delay  rst=off  infoeditControl=Selection of Reset will increase slice count due to use of real FFs and instead of SRLs  en=off  latency=3  reg_retiming=on  dbl_ovrd=off  block_type=delay
  map1 : Subsystem  Tag=xps:bram  AncestorBlock=xps_library/Memory/shared_bram  mask{arith_type=Unsigned, addr_width=11, data_width=16, reg_prim_output=on, reg_core_output=on, optimization=Minimum_Area, data_bin_pt=0, init_vals=[40, 42, 44, 46, zeros(1,2047-4)], sample_rate=1}
      mask prompts: arith_type "Output Data Type"; addr_width "Address width"; data_width "Data Width"; reg_prim_output "Register Primitive Output"; reg_core_output "Register Core Output"; data_bin_pt "Data Binary Point"; init_vals "Initial values (simulation only)"; sample_rate "Sample rate"
      mask init:
      | shared_bram_mask;
      mask TypeOptions arith_type: Unsigned | Signed  (2's comp)
      mask TypeOptions data_width: 8 | 16 | 32 | 64 | 128
      mask TypeOptions optimization: Minimum_Area | Low_Power
  never : xbsIndex_r4/Constant  const=0  gui_display_data_type=Fixed-point  arith_type=Boolean  n_bits=16  bin_pt=14  preci_type=Single  exp_width=8  frac_width=24  explicit_period=on  period=1  equ=P=C  opselect=C  inp2=PCIN>>17  opr=+  inp1=P  carry=CIN  dbl_ovrd=off  block_type=constant
  post_sync_delay : xbsIndex_r4/Delay  rst=off  infoeditControl=Selection of Reset will increase slice count due to use of real FFs and instead of SRLs  en=off  latency=4  reg_retiming=on  dbl_ovrd=off  block_type=delay
  pre_sync_delay : xbsIndex_r4/Delay  rst=off  infoeditControl=Selection of Reset will increase slice count due to use of real FFs and instead of SRLs  en=off  latency=3  reg_retiming=on  dbl_ovrd=off  block_type=delay
  sw_bram_slice : xbsIndex_r4/Slice  nbits=11  boolean_output=off  mode=Lower Bit Location + Width  bit1=0  base1=MSB of Input  bit0=0  base0=LSB of Input  dbl_ovrd=off  block_type=slice
  sync_delay : xbsIndex_r4/Delay  rst=off  infoeditControl=Selection of Reset will increase slice count due to use of real FFs and instead of SRLs  en=off  latency=2048  reg_retiming=on  dbl_ovrd=off  block_type=delay
  zero : xbsIndex_r4/Constant  const=0  gui_display_data_type=Fixed-point  arith_type=Unsigned  n_bits=16  bin_pt=0  preci_type=Single  exp_width=8  frac_width=24  explicit_period=on  period=1  equ=P=C  opselect=C  inp2=PCIN>>17  opr=+  inp1=P  carry=CIN  dbl_ovrd=off  block_type=constant
  sync_out : Outport
  dout0 : Outport  Port=2
  wires:
  sync/1 -> pre_sync_delay/1, Counter1/1
  map1/1(data_out) -> sw_bram_slice/1
  delay_sel/1 -> dbl_buffer0/1(rw_mode)
  Constant2/1 -> dbl_buffer0/5(we)
  dbl_buffer0/1(dout) -> dout0/1
  delay_d0/1 -> dbl_buffer0/2(wr_addr)
  never/1 -> map1/3(we)
  zero/1 -> map1/2(data_in)
  delay_din0/1 -> dbl_buffer0/4(din1)
  Counter1/1 -> Slice1/1, Slice2/1
  Slice1/1 -> delay_sel/1
  din0/1 -> delay_din0/1
  post_sync_delay/1 -> sync_out/1
  Slice2/1 -> delay_d0/1, map1/1(addr)
  sw_bram_slice/1 -> dbl_buffer0/3(rd_addr)
  pre_sync_delay/1 -> sync_delay/1
  sync_delay/1 -> post_sync_delay/1

== system sparrow_albatros_spec_withgpio_bram/pack_rst ==
  sim_1 : Inport
  convert1_1 : DataTypeConversion  OutDataTypeStr=fixdt('ufix1_En0')  LockScale=on
  convert2_1 : DataTypeConversion  OutDataTypeStr=fixdt('ufix1_En0')  ConvertRealWorld=Stored Integer (SI)  LockScale=on
  gain_1 : Gain  OutDataTypeStr=fixdt('ufix32_En0')
  io_delay : xbsIndex_r4/Delay  rst=off  infoeditControl=Selection of Reset will increase slice count due to use of real FFs and instead of SRLs  en=off  latency=0  reg_retiming=on  dbl_ovrd=off  block_type=delay
  slice_reg : xbsIndex_r4/Slice  nbits=1  boolean_output=on  mode=Lower Bit Location + Width  bit1=0  base1=MSB of Input  bit0=0  base0=LSB of Input  dbl_ovrd=off  block_type=slice
  sparrow_albatros_spec_withgpio_bram_pack_rst_user_data_out : xbsIndex_r4/Gateway In  gui_display_data_type=Fixed-point  arith_type=Unsigned  n_bits=32  bin_pt=0  preci_type=Single  exp_width=8  frac_width=24  rows=1  columns=1  quantization="Round  (unbiased: +/- Inf)"  overflow=Saturate  period=1  UseAsADC=off  ADCChannel='1'  interface=None  automatic_assignment=on  address_offset=hex2dec('00')  intf_name=''  intf_description=''  default_value=0  timing_constraint=None  locs_specified=off  LOCs={}  io_standard={}  inherit_from_input=off  hdl_port=on  dbl_ovrd=off  block_type=gatewayin
  in_reg : Outport
  wires:
  sparrow_albatros_spec_withgpio_bram_pack_rst_user_data_out/1 -> io_delay/1
  sim_1/1 -> convert1_1/1
  convert1_1/1 -> convert2_1/1
  convert2_1/1 -> gain_1/1
  gain_1/1 -> sparrow_albatros_spec_withgpio_bram_pack_rst_user_data_out/1
  io_delay/1 -> slice_reg/1
  slice_reg/1 -> in_reg/1
